simulink model "linear_model_alternative"  (R2023b)
settings: Solver=VariableStepAuto  StartTime=0.0  StopTime=10.0  RelTol=1e-3
undefined symbols (not defined in the file): A, B, C, D
settings Model: Creator=USER  LastModifiedBy=USER

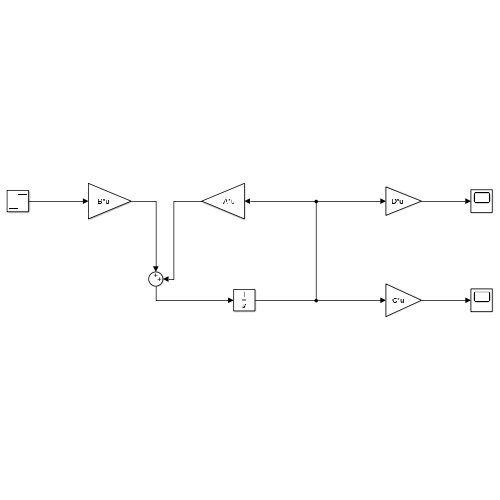
[thumbnail: Simulink's stored preview of the top-level diagram]
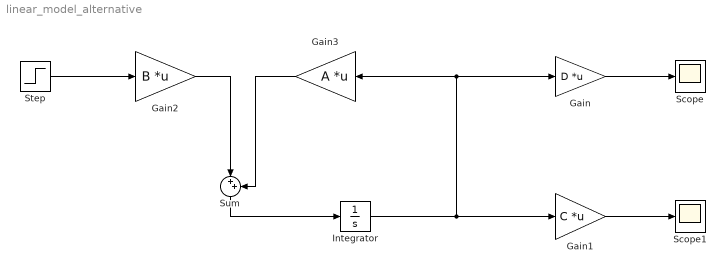
== system linear_model_alternative ==
  Gain : Gain  Gain=D  Multiplication=Matrix(K*u)
  Gain1 : Gain  Gain=C  Multiplication=Matrix(K*u)
  Gain2 : Gain  Gain=B  Multiplication=Matrix(K*u)
  Gain3 : Gain  Gain=A  Multiplication=Matrix(K*u)
  Integrator : Integrator
  Scope : Scope
  Scope1 : Scope
  Step : Step  After=10*pi/180  SampleTime=0
  Sum : Sum  Inputs=|++
  wires:
  Gain3/1 -> Sum/2
  Gain2/1 -> Sum/1
  Sum/1 -> Integrator/1
  Gain/1 -> Scope/1
  Integrator/1 -> Gain3/1, Gain/1, Gain1/1
  Gain1/1 -> Scope1/1
  Step/1 -> Gain2/1
